simulink model "openLoop"  (R2023b)
settings: Solver=FixedStepAuto  StartTime=0.0  StopTime=inf  FixedStep=0.01  RelTol=1e-3
model workspace (MAT data in the model file):
  freq = 0.87
settings Model: Creator=marko  LastModifiedBy=marko
settings DebuggingCC: UnconnectedInputMsg=warning  UnconnectedOutputMsg=warning  UnconnectedLineMsg=warning
settings ModelReferenceCC: EnableRefExpFcnMdlSchedulingChecks=on
settings RTWCC: DLArmComputeVersion=19.05

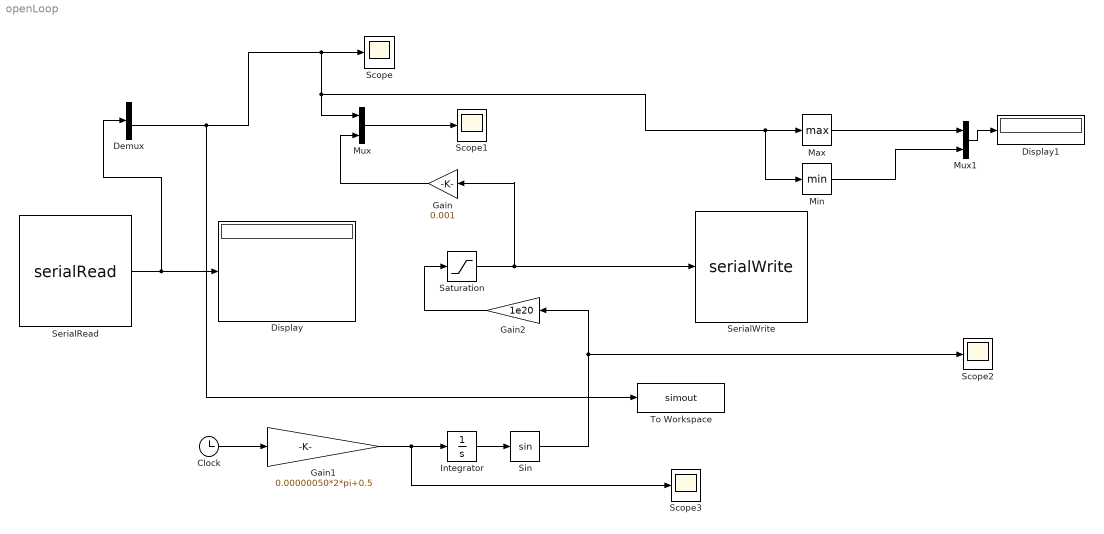
== system openLoop ==
  Clock : Clock
  Demux : Demux
  Display : Display
  Display1 : Display
  Gain : Gain  Gain=0.001
  Gain1 : Gain  Gain=0.00000050*2*pi+0.5
  Gain2 : Gain  Gain=1e20
  Integrator : Integrator
  Max : MinMax  Function=max
  Min : MinMax
  Mux : Mux  Inputs=2
  Mux1 : Mux  Inputs=2
  Saturation : Saturate  UpperLimit=4000  LowerLimit=-4000
  Scope{,1..3} (4 alike) : Scope
  SerialRead : M-S-Function  FunctionName=serialRead  Parameters='COM16'
      mask Display: image('vga2.png');
  SerialWrite : M-S-Function  FunctionName=serialWrite  Parameters='COM16'
      mask Display: image('vga3.png');
  Sin : Trigonometry
  To Workspace : ToWorkspace  VariableName=simout  SampleTime=-1
      settings: Save2DSignal=2-D array (concatenate along first dimension)
  wires:
  SerialRead/1 -> Demux/1, Display/1
  Demux/3 -> To Workspace/1, Min/1, Max/1, Mux/1, Scope/1
  Mux/1 -> Scope1/1
  Gain/1 -> Mux/2
  Saturation/1 -> Gain/1, SerialWrite/1
  Max/1 -> Mux1/1
  Min/1 -> Mux1/2
  Mux1/1 -> Display1/1
  Clock/1 -> Gain1/1
  Gain1/1 -> Scope3/1, Integrator/1
  Gain2/1 -> Saturation/1
  Integrator/1 -> Sin/1
  Sin/1 -> Scope2/1, Gain2/1
